simulink model "Tarea3"  (R2023b)
settings: Solver=VariableStepAuto  StartTime=0.0  StopTime=10  MaxStep=0.01  RelTol=1e-3
values from neighbouring files (symbols this model uses):
  A = [0 1 ... (first row only)    [ParametrosMotor.m]
  b = 0.01    [ParametrosMotor.m]
  B = [0 , 0;k/(J*R), -1/J]    [ParametrosMotor.m]
  C = [1,0;0,1]    [ParametrosMotor.m]
  g = 9.8    [ParametrosMotor.m]
  J = 42.51    [ParametrosMotor.m]
  k = 0.149    [ParametrosMotor.m]
  kd = 1    [ParametrosMotor.m]
  kp = 1    [ParametrosMotor.m]
  l = 0.05    [ParametrosMotor.m]
  m = 50    [ParametrosMotor.m]
  R = 6    [ParametrosMotor.m]
settings Model: Creator=sslan  LastModifiedBy=sslan

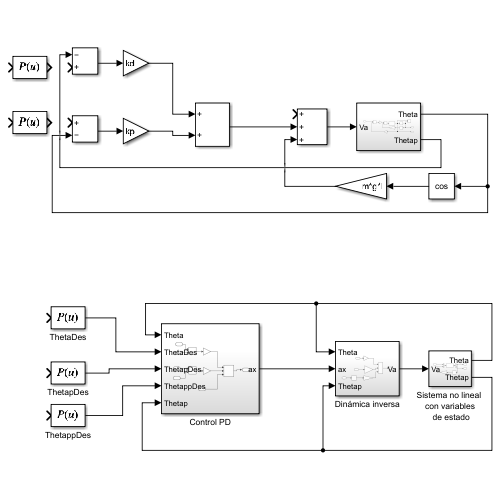
[thumbnail: Simulink's stored preview of the top-level diagram]
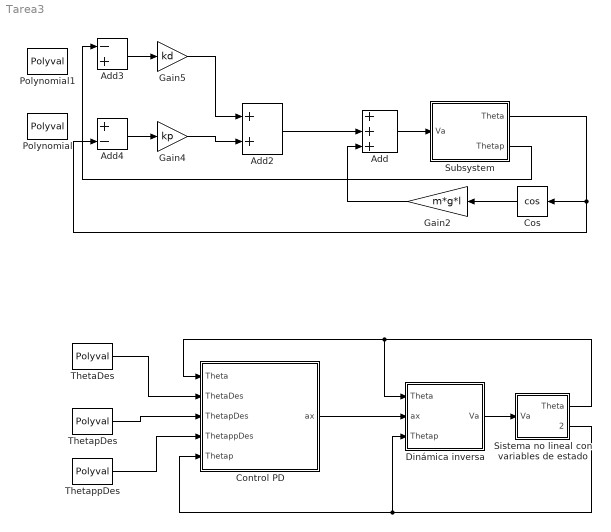
== system Tarea3 ==
  Add : Sum  Inputs=+++
  Add2 : Sum
  Add3 : Sum  Inputs=-+
  Add4 : Sum  Inputs=+-
  Control PD : Subsystem
  Cos : Trigonometry  Operator=cos
  Dinámica inversa : Subsystem
  Gain2 : Gain  Gain=m*g*l
  Gain4 : Gain  Gain=kp
  Gain5 : Gain  Gain=kd
  Polynomial : Polyval  Coefs=[ +2.081618890e-019, -1.441693666e-014, +4.719686976e-010, -8.536869453e-006, +1.621573104e-001, -8.087801117e+001 ]
  Polynomial1 : Polyval  Coefs=[ +2.081618890e-019, -1.441693666e-014, +4.719686976e-010, -8.536869453e-006, +1.621573104e-001, -8.087801117e+001 ]
  Sistema no lineal con variables de estado : Subsystem
  Subsystem : Subsystem
  ThetaDes : Polyval  Coefs=[ +2.081618890e-019, -1.441693666e-014, +4.719686976e-010, -8.536869453e-006, +1.621573104e-001, -8.087801117e+001 ]
  ThetapDes : Polyval  Coefs=[ +2.081618890e-019, -1.441693666e-014, +4.719686976e-010, -8.536869453e-006, +1.621573104e-001, -8.087801117e+001 ]
  ThetappDes : Polyval  Coefs=[ +2.081618890e-019, -1.441693666e-014, +4.719686976e-010, -8.536869453e-006, +1.621573104e-001, -8.087801117e+001 ]
  wires:
  Add4/1 -> Gain4/1
  Add3/1 -> Gain5/1
  Gain4/1 -> Add2/2
  Gain5/1 -> Add2/1
  Cos/1 -> Gain2/1
  Subsystem/1(Theta) -> Cos/1, Add4/2
  Subsystem/2(Thetap) -> Add3/1
  Gain2/1 -> Add/3
  Add2/1 -> Add/2
  Add/1 -> Subsystem/1(Va)
  Dinámica inversa/1(Va) -> Sistema no lineal con variables de estado/1(Va)
  Control PD/1(ax) -> Dinámica inversa/2(ax)
  ThetappDes/1 -> Control PD/4(ThetappDes)
  ThetapDes/1 -> Control PD/3(ThetapDes)
  ThetaDes/1 -> Control PD/2(ThetaDes)
  Sistema no lineal con variables de estado/1(Theta) -> Dinámica inversa/1(Theta), Control PD/1(Theta)
  Sistema no lineal con variables de estado/2(Thetap) -> Dinámica inversa/3(Thetap), Control PD/5(Thetap)

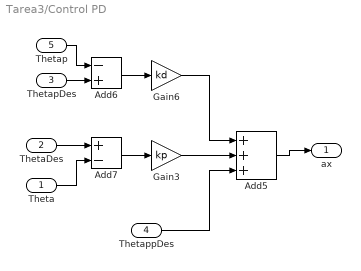
== system Tarea3/Control PD ==
  Theta : Inport
  ThetaDes : Inport  Port=2
  ThetapDes : Inport  Port=3
  ThetappDes : Inport  Port=4
  Thetap : Inport  Port=5
  Add5 : Sum  Inputs=+++
  Add6 : Sum  Inputs=-+
  Add7 : Sum  Inputs=+-
  Gain3 : Gain  Gain=kp
  Gain6 : Gain  Gain=kd
  ax : Outport
  wires:
  ThetappDes/1 -> Add5/3
  Add6/1 -> Gain6/1
  Add5/1 -> ax/1
  ThetaDes/1 -> Add7/1
  Gain3/1 -> Add5/2
  Add7/1 -> Gain3/1
  Gain6/1 -> Add5/1
  ThetapDes/1 -> Add6/2
  Thetap/1 -> Add6/1
  Theta/1 -> Add7/2

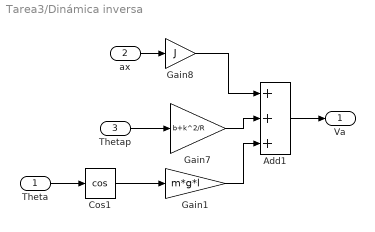
== system Tarea3/Dinámica inversa ==
  Theta : Inport
  ax : Inport  Port=2
  Thetap : Inport  Port=3
  Add1 : Sum  Inputs=+++
  Cos1 : Trigonometry  Operator=cos
  Gain1 : Gain  Gain=m*g*l
  Gain7 : Gain  Gain=b+k^2/R
  Gain8 : Gain  Gain=J
  Va : Outport
  wires:
  Theta/1 -> Cos1/1
  ax/1 -> Gain8/1
  Add1/1 -> Va/1
  Gain7/1 -> Add1/2
  Cos1/1 -> Gain1/1
  Gain1/1 -> Add1/3
  Thetap/1 -> Gain7/1
  Gain8/1 -> Add1/1

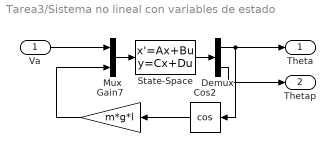
== system Tarea3/Sistema no lineal con variables de estado ==
  Va : Inport
  Cos2 : Trigonometry  Operator=cos
  Demux : Demux  Outputs=2
  Gain7 : Gain  Gain=m*g*l
  Mux : Mux  Inputs=2
  State-Space : StateSpace  A=A  B=B  C=C  D=zeros(2,2)  InitialCondition=0
  Theta : Outport
  Thetap : Outport  Port=2
  wires:
  Demux/1 -> Theta/1, Cos2/1
  State-Space/1 -> Demux/1
  Cos2/1 -> Gain7/1
  Gain7/1 -> Mux/2
  Va/1 -> Mux/1
  Mux/1 -> State-Space/1
  Demux/2 -> Thetap/1

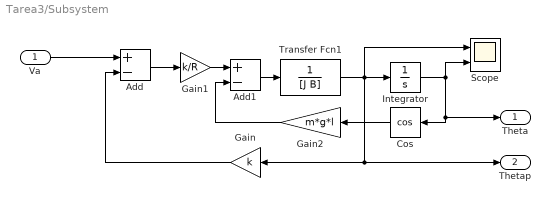
== system Tarea3/Subsystem ==
  Va : Inport
  Add : Sum  Inputs=+-
  Add1 : Sum  Inputs=+-
  Cos : Trigonometry  Operator=cos
  Gain : Gain  Gain=k
  Gain1 : Gain  Gain=k/R
  Gain2 : Gain  Gain=m*g*l
  Integrator : Integrator
  Scope : Scope  NumInputPorts=2
  Transfer Fcn1 : TransferFcn  Denominator=[J B]
  Theta : Outport
  Thetap : Outport  Port=2
  wires:
  Add/1 -> Gain1/1
  Transfer Fcn1/1 -> Scope/1, Thetap/1, Gain/1, Integrator/1
  Cos/1 -> Gain2/1
  Gain2/1 -> Add1/2
  Gain1/1 -> Add1/1
  Gain/1 -> Add/2
  Integrator/1 -> Theta/1, Cos/1, Scope/2
  Add1/1 -> Transfer Fcn1/1
  Va/1 -> Add/1
